simulink model "task4"  (R2024b)
settings: Solver=VariableStepAuto  StartTime=0.0  StopTime=10.0  RelTol=1e-3
settings Model: Creator=33657  LastModifiedBy=33657

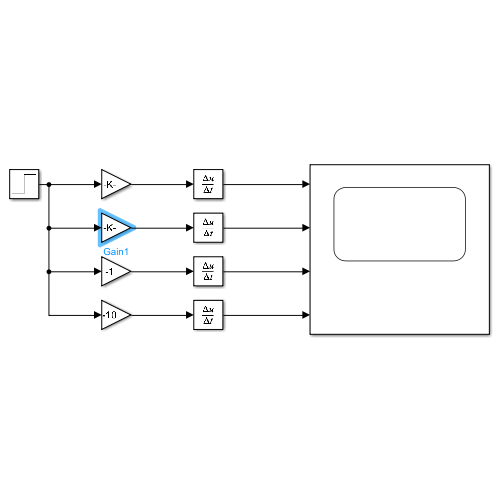
[thumbnail: Simulink's stored preview of the top-level diagram]
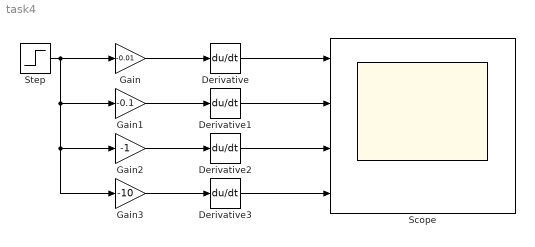
== system task4 ==
  Derivative{,1..3} (4 alike) : Derivative
  Gain : Gain  Gain=-0.01
  Gain1 : Gain  Gain=-0.1
  Gain2 : Gain  Gain=-1
  Gain3 : Gain  Gain=-10
  Scope : Scope  NumInputPorts=4
  Step : Step  SampleTime=0
  wires:
  Step/1 -> Gain3/1, Gain2/1, Gain1/1, Gain/1
  Gain/1 -> Derivative/1
  Gain1/1 -> Derivative1/1
  Gain2/1 -> Derivative2/1
  Gain3/1 -> Derivative3/1
  Derivative/1 -> Scope/1
  Derivative1/1 -> Scope/2
  Derivative2/1 -> Scope/3
  Derivative3/1 -> Scope/4
